simulink model "H02_ERR"  (R2026a)
settings: Solver=VariableStepAuto
settings Model: Creator=Szalay  LastModifiedBy=Szalay

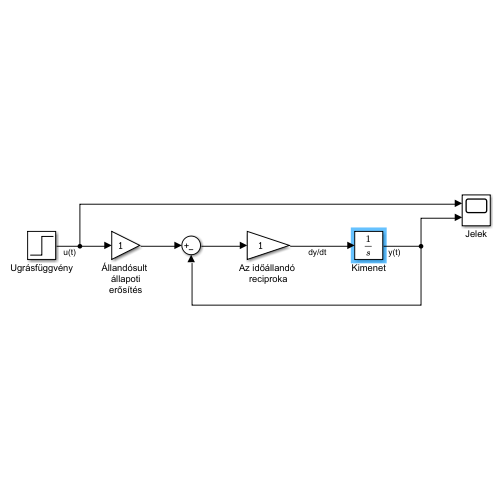
[thumbnail: Simulink's stored preview of the top-level diagram]
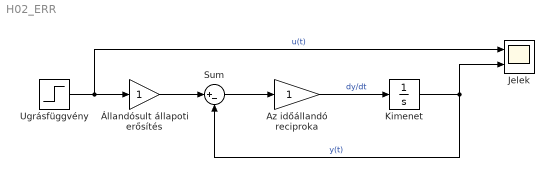
== system H02_ERR ==
  Az időállandó reciproka : Gain
  Jelek : Scope  NumInputPorts=2
      settings: ActiveDisplayYMinimum=-0.12499999999999997  ActiveDisplayYMaximum=1.125
  Kimenet : Integrator  InitialCondition=0.5
  Sum : Sum  Inputs=|+-
  Ugrásfüggvény : Step  Time=5  SampleTime=0
  Állandósult állapoti erősítés : Gain
  wires:
  Kimenet/1 -> Sum/2, Jelek/2  "y(t)"
  Az időállandó reciproka/1 -> Kimenet/1  "dy/dt"
  Sum/1 -> Az időállandó reciproka/1
  Állandósult állapoti erősítés/1 -> Sum/1
  Ugrásfüggvény/1 -> Jelek/1, Állandósult állapoti erősítés/1  "u(t)"
